simulink library "three_phase_bridge_three_level_ttype_mos_simple_2th"  (R2026a)
settings: Solver=VariableStepAuto
libraries: fl_lib x192, nesl_utility x120, mos_simple_2th_lib x12
(part 2 of 4)

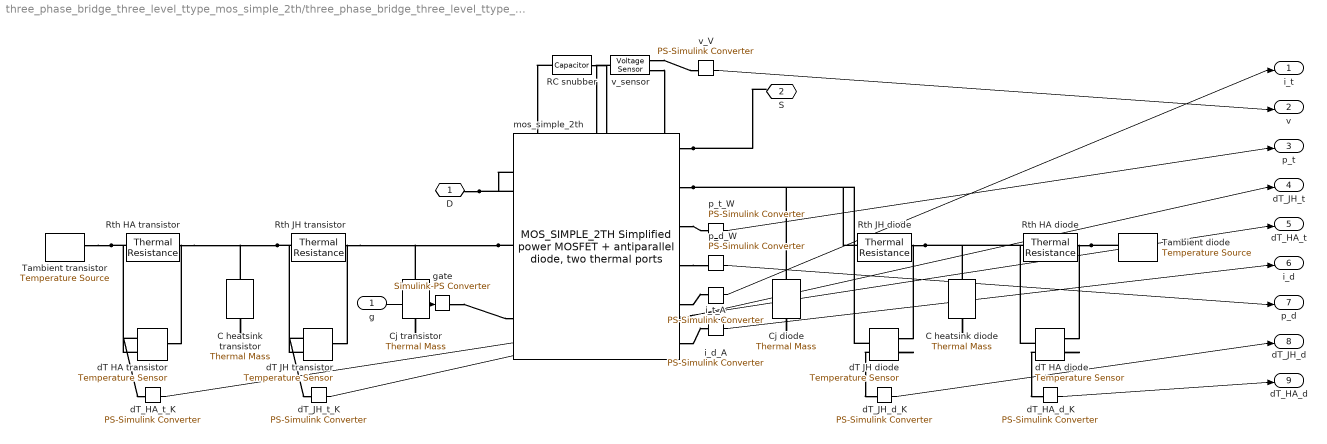
== system three_phase_bridge_three_level_ttype_mos_simple_2th/three_phase_bridge_three_level_ttype_mos_simple_2th/Q4 ==
  g : Inport
  gate : nesl_utility/Simulink-PS Converter  PhysicalDomain=network_engine_domain  SubClassName=ps_input  LeftPortType=input  RightPortType=output  PseudoPeriodic=off  Frequencies=[]  NoiseDistribution=none  NoiseParameters=[]  Unit=1  AffineConversion=off  FilteringAndDerivatives=provide  SimscapeFilterOrder=1  InputFilterTimeConstant=0.001  UdotUserProvided=0
  mos_simple_2th : mos_simple_2th_lib/MOS_SIMPLE_2TH Simplified power MOSFET + antiparallel diode, two thermal ports  Rds_on=rds_on_m mOhm  alpha_R=alpha_R_m 1/K  Tj_ref=Tj_ref_m degC  Roff=Roff_m Ohm  Vf=v_gamma_m V  Rd=rd_on_m mOhm  two_die=two_die_m  G_th=G_th_m  Eon_ref=Eon_m mJ  Eoff_ref=Eoff_m mJ  Err_ref=Err_m mJ  Iref=Ic_ref_m A  Vref=Vdc_ref_m V  ki=ki_m  kv=kv_m  Vth_off=Vth_off_m V  Vth_on=Vth_on_m V  V_sm=V_sm_m V  tau_s=time_constant_edge_m us  tau_v=tau_v_m us  tau_p=time_constant_ploss_m us  i_eps=i_eps_m A  v_eps=1e-3 V  v_specify=off  v_priority=None  v=0 V  v_nominal_specify=off  v_nominal_value=1  v_nominal_unit=V  i_specify=off  i_priority=None  i=0 A  i_nominal_specify=off  i_nominal_value=1  i_nominal_unit=A  ich_specify=off  ich_priority=None  ich=0 A  ich_nominal_specify=off  ich_nominal_value=1  ich_nominal_unit=A  ichp_specify=off  ichp_priority=None  ichp=0 A  ichp_nominal_specify=off  ichp_nominal_value=1  ichp_nominal_unit=A  idio_specify=off  idio_priority=None  idio=0 A  idio_nominal_specify=off  idio_nominal_value=1  idio_nominal_unit=A  vfd_specify=off  vfd_priority=None  vfd=0 V  vfd_nominal_specify=off  vfd_nominal_value=1  vfd_nominal_unit=V  ith_specify=off  ith_priority=None  ith=0 A  ith_nominal_specify=off  ith_nominal_value=1  ith_nominal_unit=A  idh_specify=off  idh_priority=None  idh=0 A  idh_nominal_specify=off  idh_nominal_value=1  idh_nominal_unit=A  vbl_specify=off  vbl_priority=None  vbl=600 V  vbl_nominal_specify=off  vbl_nominal_value=1  vbl_nominal_unit=V  hb_specify=off  hb_priority=None  hb=0  hb_nominal_specify=off  hb_nominal_value=1  hb_nominal_unit=1  Gch_specify=off  Gch_priority=None  Gch=0 S  Gch_nominal_specify=off  Gch_nominal_value=1  Gch_nominal_unit=S  gl_specify=off  gl_priority=None  gl=0  gl_nominal_specify=off  gl_nominal_value=1  gl_nominal_unit=1  Rds_specify=off  Rds_priority=None  Rds=1e-3 Ohm  Rds_nominal_specify=off  Rds_nominal_value=1  Rds_nominal_unit=Ohm  xr_specify=off  xr_priority=None  xr=1  xr_nominal_specify=off  xr_nominal_value=1  xr_nominal_unit=1  Eot_specify=off  Eot_priority=None  Eot=0 J  Eot_nominal_specify=off  Eot_nominal_value=1  Eot_nominal_unit=J  Eod_specify=off  Eod_priority=None  Eod=0 J  Eod_nominal_specify=off  Eod_nominal_value=1  Eod_nominal_unit=J  Pswt_specify=off  Pswt_priority=None  Pswt=0 W  Pswt_nominal_specify=off  Pswt_nominal_value=1  Pswt_nominal_unit=W  Pswd_specify=off  Pswd_priority=None  Pswd=0 W  Pswd_nominal_specify=off  Pswd_nominal_value=1  Pswd_nominal_unit=W  Pct_specify=off  Pct_priority=None  Pct=0 W  Pct_nominal_specify=off  Pct_nominal_value=1  Pct_nominal_unit=W  Pcd_specify=off  Pcd_priority=None  Pcd=0 W  Pcd_nominal_specify=off  Pcd_nominal_value=1  Pcd_nominal_unit=W  Qt_specify=off  Qt_priority=None  Qt=0 W  Qt_nominal_specify=off  Qt_nominal_value=1  Qt_nominal_unit=W  Qd_specify=off  Qd_priority=None  Qd=0 W  Qd_nominal_specify=off  Qd_nominal_value=1  Qd_nominal_unit=W  Eqt_specify=off  Eqt_priority=None  Eqt=0 J  Eqd_specify=off  Eqd_priority=None  Eqd=0 J
  D : PMIOPort  Side=Left
  S : PMIOPort  Port=2  Side=Right
  RC snubber : fl_lib/Electrical/Electrical Elements/Capacitor  c=Csnubber_m F  r=Rsnubber_m Ohm  g=0 1/Ohm  i_specify=off  i_priority=None  i=0 A  i_nominal_specify=off  i_nominal_value=1  i_nominal_unit=A  v_specify=off  v_priority=None  v=0 V  v_nominal_specify=off  v_nominal_value=1  v_nominal_unit=V  vc_specify=off  vc_priority=High  vc=0 V  vc_nominal_specify=off  vc_nominal_value=1  vc_nominal_unit=V
  v_sensor : fl_lib/Electrical/Electrical Sensors/Voltage Sensor
  v_V : nesl_utility/PS-Simulink Converter  PhysicalDomain=network_engine_domain  SubClassName=ps_output  LeftPortType=input  RightPortType=output  PseudoPeriodic=off  Frequencies=[]  VectorFormat=1-D array  Unit=V  AffineConversion=off
  p_t_W : nesl_utility/PS-Simulink Converter  PhysicalDomain=network_engine_domain  SubClassName=ps_output  LeftPortType=input  RightPortType=output  PseudoPeriodic=off  Frequencies=[]  VectorFormat=1-D array  Unit=W  AffineConversion=off
  p_d_W : nesl_utility/PS-Simulink Converter  PhysicalDomain=network_engine_domain  SubClassName=ps_output  LeftPortType=input  RightPortType=output  PseudoPeriodic=off  Frequencies=[]  VectorFormat=1-D array  Unit=W  AffineConversion=off
  i_t_A : nesl_utility/PS-Simulink Converter  PhysicalDomain=network_engine_domain  SubClassName=ps_output  LeftPortType=input  RightPortType=output  PseudoPeriodic=off  Frequencies=[]  VectorFormat=1-D array  Unit=A  AffineConversion=off
  i_d_A : nesl_utility/PS-Simulink Converter  PhysicalDomain=network_engine_domain  SubClassName=ps_output  LeftPortType=input  RightPortType=output  PseudoPeriodic=off  Frequencies=[]  VectorFormat=1-D array  Unit=A  AffineConversion=off
  Cj transistor : fl_lib/Thermal/Thermal Elements/Thermal Mass  mass_type=foundation.enum.constant_variable.constant  mass=JunctionTermalMass_m/specific_heat_m kg  sp_heat=specific_heat_m J/(K*kg)  mass_min=1e-6 kg  num_ports=foundation.enum.numPorts2.one  m_specify=off  m_priority=High  m=1 kg  m_nominal_specify=off  m_nominal_value=1  m_nominal_unit=kg  T_specify=on  T_priority=High  T=Tambient_m degC  T_nominal_specify=off  T_nominal_value=1  T_nominal_unit=K  Q_specify=off  Q_priority=High  Q=0 W  Q_nominal_specify=off  Q_nominal_value=1  Q_nominal_unit=W
  Rth JH transistor : fl_lib/Thermal/Thermal Elements/Thermal Resistance  resistance=rth_switch_JH_m K/W  T_specify=off  T_priority=High  T=0 deltadegC  T_nominal_specify=off  T_nominal_value=1  T_nominal_unit=K  Q_specify=off  Q_priority=None  Q=0 W  Q_nominal_specify=off  Q_nominal_value=1  Q_nominal_unit=W
  C heatsink transistor : fl_lib/Thermal/Thermal Elements/Thermal Mass  mass_type=foundation.enum.constant_variable.constant  mass=mass_heatsink_m kg  sp_heat=specific_heat_m J/(K*kg)  mass_min=1e-6 kg  num_ports=foundation.enum.numPorts2.one  m_specify=off  m_priority=High  m=1 kg  m_nominal_specify=off  m_nominal_value=1  m_nominal_unit=kg  T_specify=on  T_priority=High  T=Tambient_m degC  T_nominal_specify=off  T_nominal_value=1  T_nominal_unit=K  Q_specify=off  Q_priority=High  Q=0 W  Q_nominal_specify=off  Q_nominal_value=1  Q_nominal_unit=W
  Rth HA transistor : fl_lib/Thermal/Thermal Elements/Thermal Resistance  resistance=rth_switch_HA_m K/W  T_specify=off  T_priority=High  T=0 deltadegC  T_nominal_specify=off  T_nominal_value=1  T_nominal_unit=K  Q_specify=off  Q_priority=None  Q=0 W  Q_nominal_specify=off  Q_nominal_value=1  Q_nominal_unit=W
  Tambient transistor : fl_lib/Thermal/Thermal Sources/Temperature Source  temperature=Tambient_m degC
  dT JH transistor : fl_lib/Thermal/Thermal Sensors/Temperature Sensor  temperature_measure=foundation.enum.MeasurementReference.difference
  dT HA transistor : fl_lib/Thermal/Thermal Sensors/Temperature Sensor  temperature_measure=foundation.enum.MeasurementReference.difference
  dT_JH_t_K : nesl_utility/PS-Simulink Converter  PhysicalDomain=network_engine_domain  SubClassName=ps_output  LeftPortType=input  RightPortType=output  PseudoPeriodic=off  Frequencies=[]  VectorFormat=1-D array  Unit=K  AffineConversion=off
  dT_HA_t_K : nesl_utility/PS-Simulink Converter  PhysicalDomain=network_engine_domain  SubClassName=ps_output  LeftPortType=input  RightPortType=output  PseudoPeriodic=off  Frequencies=[]  VectorFormat=1-D array  Unit=K  AffineConversion=off
  Cj diode : fl_lib/Thermal/Thermal Elements/Thermal Mass  mass_type=foundation.enum.constant_variable.constant  mass=JunctionTermalMass_m/specific_heat_m kg  sp_heat=specific_heat_m J/(K*kg)  mass_min=1e-6 kg  num_ports=foundation.enum.numPorts2.one  m_specify=off  m_priority=High  m=1 kg  m_nominal_specify=off  m_nominal_value=1  m_nominal_unit=kg  T_specify=on  T_priority=High  T=Tambient_m degC  T_nominal_specify=off  T_nominal_value=1  T_nominal_unit=K  Q_specify=off  Q_priority=High  Q=0 W  Q_nominal_specify=off  Q_nominal_value=1  Q_nominal_unit=W
  Rth JH diode : fl_lib/Thermal/Thermal Elements/Thermal Resistance  resistance=rth_diode_JH_m K/W  T_specify=off  T_priority=High  T=0 deltadegC  T_nominal_specify=off  T_nominal_value=1  T_nominal_unit=K  Q_specify=off  Q_priority=None  Q=0 W  Q_nominal_specify=off  Q_nominal_value=1  Q_nominal_unit=W
  C heatsink diode : fl_lib/Thermal/Thermal Elements/Thermal Mass  mass_type=foundation.enum.constant_variable.constant  mass=mass_heatsink_m kg  sp_heat=specific_heat_m J/(K*kg)  mass_min=1e-6 kg  num_ports=foundation.enum.numPorts2.one  m_specify=off  m_priority=High  m=1 kg  m_nominal_specify=off  m_nominal_value=1  m_nominal_unit=kg  T_specify=on  T_priority=High  T=Tambient_m degC  T_nominal_specify=off  T_nominal_value=1  T_nominal_unit=K  Q_specify=off  Q_priority=High  Q=0 W  Q_nominal_specify=off  Q_nominal_value=1  Q_nominal_unit=W
  Rth HA diode : fl_lib/Thermal/Thermal Elements/Thermal Resistance  resistance=rth_diode_HA_m K/W  T_specify=off  T_priority=High  T=0 deltadegC  T_nominal_specify=off  T_nominal_value=1  T_nominal_unit=K  Q_specify=off  Q_priority=None  Q=0 W  Q_nominal_specify=off  Q_nominal_value=1  Q_nominal_unit=W
  Tambient diode : fl_lib/Thermal/Thermal Sources/Temperature Source  temperature=Tambient_m degC
  dT JH diode : fl_lib/Thermal/Thermal Sensors/Temperature Sensor  temperature_measure=foundation.enum.MeasurementReference.difference
  dT HA diode : fl_lib/Thermal/Thermal Sensors/Temperature Sensor  temperature_measure=foundation.enum.MeasurementReference.difference
  dT_JH_d_K : nesl_utility/PS-Simulink Converter  PhysicalDomain=network_engine_domain  SubClassName=ps_output  LeftPortType=input  RightPortType=output  PseudoPeriodic=off  Frequencies=[]  VectorFormat=1-D array  Unit=K  AffineConversion=off
  dT_HA_d_K : nesl_utility/PS-Simulink Converter  PhysicalDomain=network_engine_domain  SubClassName=ps_output  LeftPortType=input  RightPortType=output  PseudoPeriodic=off  Frequencies=[]  VectorFormat=1-D array  Unit=K  AffineConversion=off
  i_t : Outport
  v : Outport  Port=2
  p_t : Outport  Port=3
  dT_JH_t : Outport  Port=4
  dT_HA_t : Outport  Port=5
  i_d : Outport  Port=6
  p_d : Outport  Port=7
  dT_JH_d : Outport  Port=8
  dT_HA_d : Outport  Port=9
  wires:
  i_t_A/1 -> i_t/1
  v_V/1 -> v/1
  p_t_W/1 -> p_t/1
  dT_JH_t_K/1 -> dT_JH_t/1
  dT_HA_t_K/1 -> dT_HA_t/1
  i_d_A/1 -> i_d/1
  p_d_W/1 -> p_d/1
  dT_JH_d_K/1 -> dT_JH_d/1
  dT_HA_d_K/1 -> dT_HA_d/1
  g/1 -> gate/1
  connections:
  Rth JH transistor/RConn1 -- C heatsink transistor/LConn1 -- Rth HA transistor/LConn1 -- dT JH transistor/RConn1 -- dT HA transistor/LConn1
  Rth HA transistor/RConn1 -- Tambient transistor/LConn1 -- dT HA transistor/RConn1
  dT JH transistor/RConn2 -- dT_JH_t_K/LConn1
  dT HA transistor/RConn2 -- dT_HA_t_K/LConn1
  Rth JH diode/RConn1 -- C heatsink diode/LConn1 -- Rth HA diode/LConn1 -- dT JH diode/RConn1 -- dT HA diode/LConn1
  Rth HA diode/RConn1 -- Tambient diode/LConn1 -- dT HA diode/RConn1
  dT JH diode/RConn2 -- dT_JH_d_K/LConn1
  dT HA diode/RConn2 -- dT_HA_d_K/LConn1
  gate/RConn1 -- mos_simple_2th/LConn3
  D/RConn1 -- mos_simple_2th/LConn1 -- RC snubber/LConn1 -- v_sensor/LConn1
  mos_simple_2th/RConn1 -- S/RConn1 -- RC snubber/RConn1 -- v_sensor/RConn2
  v_sensor/RConn1 -- v_V/LConn1
  mos_simple_2th/RConn3 -- p_t_W/LConn1
  mos_simple_2th/RConn4 -- p_d_W/LConn1
  mos_simple_2th/RConn5 -- i_t_A/LConn1
  mos_simple_2th/RConn6 -- i_d_A/LConn1
  mos_simple_2th/LConn2 -- Cj transistor/LConn1 -- Rth JH transistor/LConn1 -- dT JH transistor/LConn1
  mos_simple_2th/RConn2 -- Cj diode/LConn1 -- Rth JH diode/LConn1 -- dT JH diode/LConn1

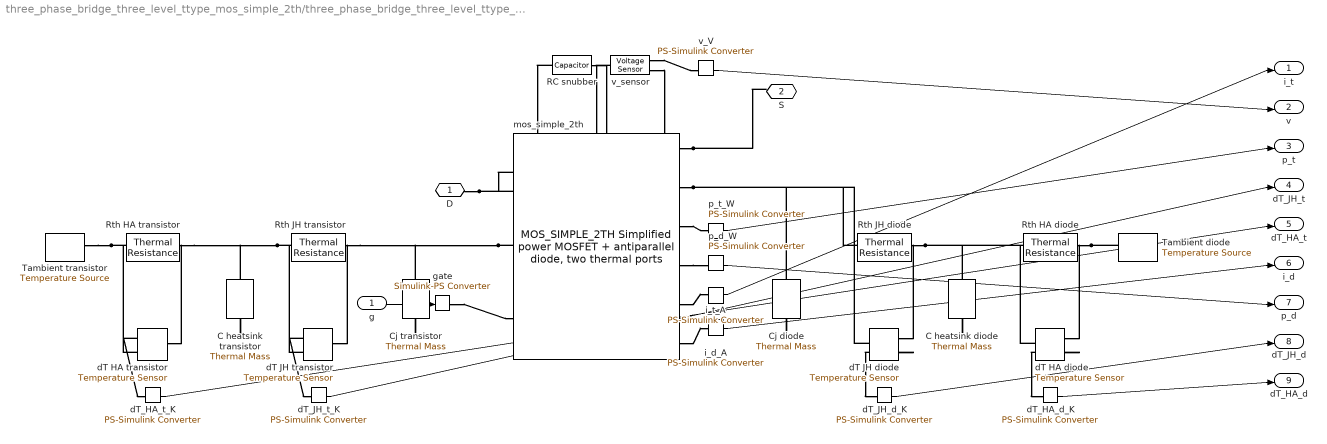
== system three_phase_bridge_three_level_ttype_mos_simple_2th/three_phase_bridge_three_level_ttype_mos_simple_2th/Q5 ==
  g : Inport
  gate : nesl_utility/Simulink-PS Converter  PhysicalDomain=network_engine_domain  SubClassName=ps_input  LeftPortType=input  RightPortType=output  PseudoPeriodic=off  Frequencies=[]  NoiseDistribution=none  NoiseParameters=[]  Unit=1  AffineConversion=off  FilteringAndDerivatives=provide  SimscapeFilterOrder=1  InputFilterTimeConstant=0.001  UdotUserProvided=0
  mos_simple_2th : mos_simple_2th_lib/MOS_SIMPLE_2TH Simplified power MOSFET + antiparallel diode, two thermal ports  Rds_on=rds_on_m mOhm  alpha_R=alpha_R_m 1/K  Tj_ref=Tj_ref_m degC  Roff=Roff_m Ohm  Vf=v_gamma_m V  Rd=rd_on_m mOhm  two_die=two_die_m  G_th=G_th_m  Eon_ref=Eon_m mJ  Eoff_ref=Eoff_m mJ  Err_ref=Err_m mJ  Iref=Ic_ref_m A  Vref=Vdc_ref_m V  ki=ki_m  kv=kv_m  Vth_off=Vth_off_m V  Vth_on=Vth_on_m V  V_sm=V_sm_m V  tau_s=time_constant_edge_m us  tau_v=tau_v_m us  tau_p=time_constant_ploss_m us  i_eps=i_eps_m A  v_eps=1e-3 V  v_specify=off  v_priority=None  v=0 V  v_nominal_specify=off  v_nominal_value=1  v_nominal_unit=V  i_specify=off  i_priority=None  i=0 A  i_nominal_specify=off  i_nominal_value=1  i_nominal_unit=A  ich_specify=off  ich_priority=None  ich=0 A  ich_nominal_specify=off  ich_nominal_value=1  ich_nominal_unit=A  ichp_specify=off  ichp_priority=None  ichp=0 A  ichp_nominal_specify=off  ichp_nominal_value=1  ichp_nominal_unit=A  idio_specify=off  idio_priority=None  idio=0 A  idio_nominal_specify=off  idio_nominal_value=1  idio_nominal_unit=A  vfd_specify=off  vfd_priority=None  vfd=0 V  vfd_nominal_specify=off  vfd_nominal_value=1  vfd_nominal_unit=V  ith_specify=off  ith_priority=None  ith=0 A  ith_nominal_specify=off  ith_nominal_value=1  ith_nominal_unit=A  idh_specify=off  idh_priority=None  idh=0 A  idh_nominal_specify=off  idh_nominal_value=1  idh_nominal_unit=A  vbl_specify=off  vbl_priority=None  vbl=600 V  vbl_nominal_specify=off  vbl_nominal_value=1  vbl_nominal_unit=V  hb_specify=off  hb_priority=None  hb=0  hb_nominal_specify=off  hb_nominal_value=1  hb_nominal_unit=1  Gch_specify=off  Gch_priority=None  Gch=0 S  Gch_nominal_specify=off  Gch_nominal_value=1  Gch_nominal_unit=S  gl_specify=off  gl_priority=None  gl=0  gl_nominal_specify=off  gl_nominal_value=1  gl_nominal_unit=1  Rds_specify=off  Rds_priority=None  Rds=1e-3 Ohm  Rds_nominal_specify=off  Rds_nominal_value=1  Rds_nominal_unit=Ohm  xr_specify=off  xr_priority=None  xr=1  xr_nominal_specify=off  xr_nominal_value=1  xr_nominal_unit=1  Eot_specify=off  Eot_priority=None  Eot=0 J  Eot_nominal_specify=off  Eot_nominal_value=1  Eot_nominal_unit=J  Eod_specify=off  Eod_priority=None  Eod=0 J  Eod_nominal_specify=off  Eod_nominal_value=1  Eod_nominal_unit=J  Pswt_specify=off  Pswt_priority=None  Pswt=0 W  Pswt_nominal_specify=off  Pswt_nominal_value=1  Pswt_nominal_unit=W  Pswd_specify=off  Pswd_priority=None  Pswd=0 W  Pswd_nominal_specify=off  Pswd_nominal_value=1  Pswd_nominal_unit=W  Pct_specify=off  Pct_priority=None  Pct=0 W  Pct_nominal_specify=off  Pct_nominal_value=1  Pct_nominal_unit=W  Pcd_specify=off  Pcd_priority=None  Pcd=0 W  Pcd_nominal_specify=off  Pcd_nominal_value=1  Pcd_nominal_unit=W  Qt_specify=off  Qt_priority=None  Qt=0 W  Qt_nominal_specify=off  Qt_nominal_value=1  Qt_nominal_unit=W  Qd_specify=off  Qd_priority=None  Qd=0 W  Qd_nominal_specify=off  Qd_nominal_value=1  Qd_nominal_unit=W  Eqt_specify=off  Eqt_priority=None  Eqt=0 J  Eqd_specify=off  Eqd_priority=None  Eqd=0 J
  D : PMIOPort  Side=Left
  S : PMIOPort  Port=2  Side=Right
  RC snubber : fl_lib/Electrical/Electrical Elements/Capacitor  c=Csnubber_m F  r=Rsnubber_m Ohm  g=0 1/Ohm  i_specify=off  i_priority=None  i=0 A  i_nominal_specify=off  i_nominal_value=1  i_nominal_unit=A  v_specify=off  v_priority=None  v=0 V  v_nominal_specify=off  v_nominal_value=1  v_nominal_unit=V  vc_specify=off  vc_priority=High  vc=0 V  vc_nominal_specify=off  vc_nominal_value=1  vc_nominal_unit=V
  v_sensor : fl_lib/Electrical/Electrical Sensors/Voltage Sensor
  v_V : nesl_utility/PS-Simulink Converter  PhysicalDomain=network_engine_domain  SubClassName=ps_output  LeftPortType=input  RightPortType=output  PseudoPeriodic=off  Frequencies=[]  VectorFormat=1-D array  Unit=V  AffineConversion=off
  p_t_W : nesl_utility/PS-Simulink Converter  PhysicalDomain=network_engine_domain  SubClassName=ps_output  LeftPortType=input  RightPortType=output  PseudoPeriodic=off  Frequencies=[]  VectorFormat=1-D array  Unit=W  AffineConversion=off
  p_d_W : nesl_utility/PS-Simulink Converter  PhysicalDomain=network_engine_domain  SubClassName=ps_output  LeftPortType=input  RightPortType=output  PseudoPeriodic=off  Frequencies=[]  VectorFormat=1-D array  Unit=W  AffineConversion=off
  i_t_A : nesl_utility/PS-Simulink Converter  PhysicalDomain=network_engine_domain  SubClassName=ps_output  LeftPortType=input  RightPortType=output  PseudoPeriodic=off  Frequencies=[]  VectorFormat=1-D array  Unit=A  AffineConversion=off
  i_d_A : nesl_utility/PS-Simulink Converter  PhysicalDomain=network_engine_domain  SubClassName=ps_output  LeftPortType=input  RightPortType=output  PseudoPeriodic=off  Frequencies=[]  VectorFormat=1-D array  Unit=A  AffineConversion=off
  Cj transistor : fl_lib/Thermal/Thermal Elements/Thermal Mass  mass_type=foundation.enum.constant_variable.constant  mass=JunctionTermalMass_m/specific_heat_m kg  sp_heat=specific_heat_m J/(K*kg)  mass_min=1e-6 kg  num_ports=foundation.enum.numPorts2.one  m_specify=off  m_priority=High  m=1 kg  m_nominal_specify=off  m_nominal_value=1  m_nominal_unit=kg  T_specify=on  T_priority=High  T=Tambient_m degC  T_nominal_specify=off  T_nominal_value=1  T_nominal_unit=K  Q_specify=off  Q_priority=High  Q=0 W  Q_nominal_specify=off  Q_nominal_value=1  Q_nominal_unit=W
  Rth JH transistor : fl_lib/Thermal/Thermal Elements/Thermal Resistance  resistance=rth_switch_JH_m K/W  T_specify=off  T_priority=High  T=0 deltadegC  T_nominal_specify=off  T_nominal_value=1  T_nominal_unit=K  Q_specify=off  Q_priority=None  Q=0 W  Q_nominal_specify=off  Q_nominal_value=1  Q_nominal_unit=W
  C heatsink transistor : fl_lib/Thermal/Thermal Elements/Thermal Mass  mass_type=foundation.enum.constant_variable.constant  mass=mass_heatsink_m kg  sp_heat=specific_heat_m J/(K*kg)  mass_min=1e-6 kg  num_ports=foundation.enum.numPorts2.one  m_specify=off  m_priority=High  m=1 kg  m_nominal_specify=off  m_nominal_value=1  m_nominal_unit=kg  T_specify=on  T_priority=High  T=Tambient_m degC  T_nominal_specify=off  T_nominal_value=1  T_nominal_unit=K  Q_specify=off  Q_priority=High  Q=0 W  Q_nominal_specify=off  Q_nominal_value=1  Q_nominal_unit=W
  Rth HA transistor : fl_lib/Thermal/Thermal Elements/Thermal Resistance  resistance=rth_switch_HA_m K/W  T_specify=off  T_priority=High  T=0 deltadegC  T_nominal_specify=off  T_nominal_value=1  T_nominal_unit=K  Q_specify=off  Q_priority=None  Q=0 W  Q_nominal_specify=off  Q_nominal_value=1  Q_nominal_unit=W
  Tambient transistor : fl_lib/Thermal/Thermal Sources/Temperature Source  temperature=Tambient_m degC
  dT JH transistor : fl_lib/Thermal/Thermal Sensors/Temperature Sensor  temperature_measure=foundation.enum.MeasurementReference.difference
  dT HA transistor : fl_lib/Thermal/Thermal Sensors/Temperature Sensor  temperature_measure=foundation.enum.MeasurementReference.difference
  dT_JH_t_K : nesl_utility/PS-Simulink Converter  PhysicalDomain=network_engine_domain  SubClassName=ps_output  LeftPortType=input  RightPortType=output  PseudoPeriodic=off  Frequencies=[]  VectorFormat=1-D array  Unit=K  AffineConversion=off
  dT_HA_t_K : nesl_utility/PS-Simulink Converter  PhysicalDomain=network_engine_domain  SubClassName=ps_output  LeftPortType=input  RightPortType=output  PseudoPeriodic=off  Frequencies=[]  VectorFormat=1-D array  Unit=K  AffineConversion=off
  Cj diode : fl_lib/Thermal/Thermal Elements/Thermal Mass  mass_type=foundation.enum.constant_variable.constant  mass=JunctionTermalMass_m/specific_heat_m kg  sp_heat=specific_heat_m J/(K*kg)  mass_min=1e-6 kg  num_ports=foundation.enum.numPorts2.one  m_specify=off  m_priority=High  m=1 kg  m_nominal_specify=off  m_nominal_value=1  m_nominal_unit=kg  T_specify=on  T_priority=High  T=Tambient_m degC  T_nominal_specify=off  T_nominal_value=1  T_nominal_unit=K  Q_specify=off  Q_priority=High  Q=0 W  Q_nominal_specify=off  Q_nominal_value=1  Q_nominal_unit=W
  Rth JH diode : fl_lib/Thermal/Thermal Elements/Thermal Resistance  resistance=rth_diode_JH_m K/W  T_specify=off  T_priority=High  T=0 deltadegC  T_nominal_specify=off  T_nominal_value=1  T_nominal_unit=K  Q_specify=off  Q_priority=None  Q=0 W  Q_nominal_specify=off  Q_nominal_value=1  Q_nominal_unit=W
  C heatsink diode : fl_lib/Thermal/Thermal Elements/Thermal Mass  mass_type=foundation.enum.constant_variable.constant  mass=mass_heatsink_m kg  sp_heat=specific_heat_m J/(K*kg)  mass_min=1e-6 kg  num_ports=foundation.enum.numPorts2.one  m_specify=off  m_priority=High  m=1 kg  m_nominal_specify=off  m_nominal_value=1  m_nominal_unit=kg  T_specify=on  T_priority=High  T=Tambient_m degC  T_nominal_specify=off  T_nominal_value=1  T_nominal_unit=K  Q_specify=off  Q_priority=High  Q=0 W  Q_nominal_specify=off  Q_nominal_value=1  Q_nominal_unit=W
  Rth HA diode : fl_lib/Thermal/Thermal Elements/Thermal Resistance  resistance=rth_diode_HA_m K/W  T_specify=off  T_priority=High  T=0 deltadegC  T_nominal_specify=off  T_nominal_value=1  T_nominal_unit=K  Q_specify=off  Q_priority=None  Q=0 W  Q_nominal_specify=off  Q_nominal_value=1  Q_nominal_unit=W
  Tambient diode : fl_lib/Thermal/Thermal Sources/Temperature Source  temperature=Tambient_m degC
  dT JH diode : fl_lib/Thermal/Thermal Sensors/Temperature Sensor  temperature_measure=foundation.enum.MeasurementReference.difference
  dT HA diode : fl_lib/Thermal/Thermal Sensors/Temperature Sensor  temperature_measure=foundation.enum.MeasurementReference.difference
  dT_JH_d_K : nesl_utility/PS-Simulink Converter  PhysicalDomain=network_engine_domain  SubClassName=ps_output  LeftPortType=input  RightPortType=output  PseudoPeriodic=off  Frequencies=[]  VectorFormat=1-D array  Unit=K  AffineConversion=off
  dT_HA_d_K : nesl_utility/PS-Simulink Converter  PhysicalDomain=network_engine_domain  SubClassName=ps_output  LeftPortType=input  RightPortType=output  PseudoPeriodic=off  Frequencies=[]  VectorFormat=1-D array  Unit=K  AffineConversion=off
  i_t : Outport
  v : Outport  Port=2
  p_t : Outport  Port=3
  dT_JH_t : Outport  Port=4
  dT_HA_t : Outport  Port=5
  i_d : Outport  Port=6
  p_d : Outport  Port=7
  dT_JH_d : Outport  Port=8
  dT_HA_d : Outport  Port=9
  wires:
  i_t_A/1 -> i_t/1
  v_V/1 -> v/1
  p_t_W/1 -> p_t/1
  dT_JH_t_K/1 -> dT_JH_t/1
  dT_HA_t_K/1 -> dT_HA_t/1
  i_d_A/1 -> i_d/1
  p_d_W/1 -> p_d/1
  dT_JH_d_K/1 -> dT_JH_d/1
  dT_HA_d_K/1 -> dT_HA_d/1
  g/1 -> gate/1
  connections:
  Rth JH transistor/RConn1 -- C heatsink transistor/LConn1 -- Rth HA transistor/LConn1 -- dT JH transistor/RConn1 -- dT HA transistor/LConn1
  Rth HA transistor/RConn1 -- Tambient transistor/LConn1 -- dT HA transistor/RConn1
  dT JH transistor/RConn2 -- dT_JH_t_K/LConn1
  dT HA transistor/RConn2 -- dT_HA_t_K/LConn1
  Rth JH diode/RConn1 -- C heatsink diode/LConn1 -- Rth HA diode/LConn1 -- dT JH diode/RConn1 -- dT HA diode/LConn1
  Rth HA diode/RConn1 -- Tambient diode/LConn1 -- dT HA diode/RConn1
  dT JH diode/RConn2 -- dT_JH_d_K/LConn1
  dT HA diode/RConn2 -- dT_HA_d_K/LConn1
  gate/RConn1 -- mos_simple_2th/LConn3
  D/RConn1 -- mos_simple_2th/LConn1 -- RC snubber/LConn1 -- v_sensor/LConn1
  mos_simple_2th/RConn1 -- S/RConn1 -- RC snubber/RConn1 -- v_sensor/RConn2
  v_sensor/RConn1 -- v_V/LConn1
  mos_simple_2th/RConn3 -- p_t_W/LConn1
  mos_simple_2th/RConn4 -- p_d_W/LConn1
  mos_simple_2th/RConn5 -- i_t_A/LConn1
  mos_simple_2th/RConn6 -- i_d_A/LConn1
  mos_simple_2th/LConn2 -- Cj transistor/LConn1 -- Rth JH transistor/LConn1 -- dT JH transistor/LConn1
  mos_simple_2th/RConn2 -- Cj diode/LConn1 -- Rth JH diode/LConn1 -- dT JH diode/LConn1

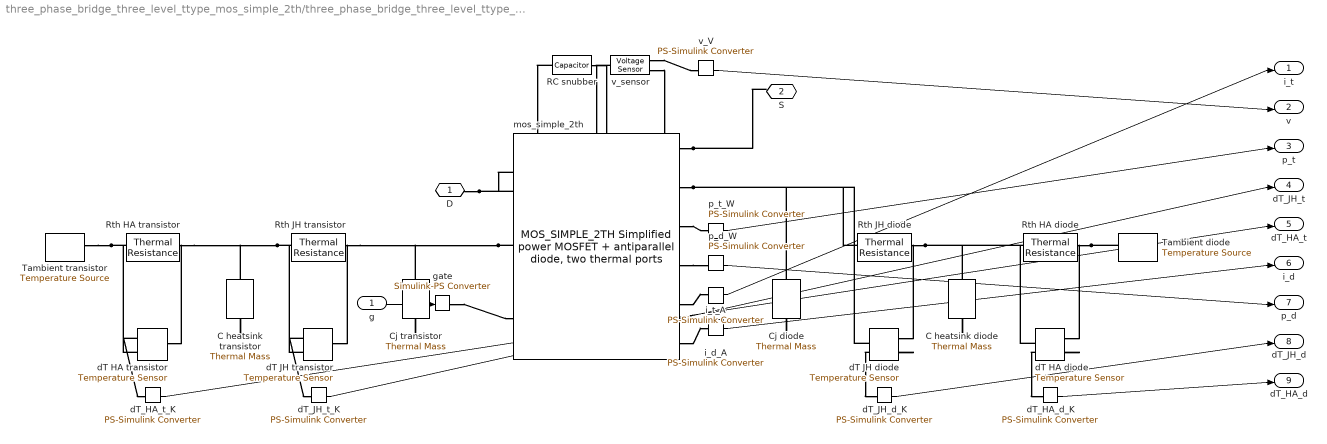
== system three_phase_bridge_three_level_ttype_mos_simple_2th/three_phase_bridge_three_level_ttype_mos_simple_2th/Q6 ==
  g : Inport
  gate : nesl_utility/Simulink-PS Converter  PhysicalDomain=network_engine_domain  SubClassName=ps_input  LeftPortType=input  RightPortType=output  PseudoPeriodic=off  Frequencies=[]  NoiseDistribution=none  NoiseParameters=[]  Unit=1  AffineConversion=off  FilteringAndDerivatives=provide  SimscapeFilterOrder=1  InputFilterTimeConstant=0.001  UdotUserProvided=0
  mos_simple_2th : mos_simple_2th_lib/MOS_SIMPLE_2TH Simplified power MOSFET + antiparallel diode, two thermal ports  Rds_on=rds_on_m mOhm  alpha_R=alpha_R_m 1/K  Tj_ref=Tj_ref_m degC  Roff=Roff_m Ohm  Vf=v_gamma_m V  Rd=rd_on_m mOhm  two_die=two_die_m  G_th=G_th_m  Eon_ref=Eon_m mJ  Eoff_ref=Eoff_m mJ  Err_ref=Err_m mJ  Iref=Ic_ref_m A  Vref=Vdc_ref_m V  ki=ki_m  kv=kv_m  Vth_off=Vth_off_m V  Vth_on=Vth_on_m V  V_sm=V_sm_m V  tau_s=time_constant_edge_m us  tau_v=tau_v_m us  tau_p=time_constant_ploss_m us  i_eps=i_eps_m A  v_eps=1e-3 V  v_specify=off  v_priority=None  v=0 V  v_nominal_specify=off  v_nominal_value=1  v_nominal_unit=V  i_specify=off  i_priority=None  i=0 A  i_nominal_specify=off  i_nominal_value=1  i_nominal_unit=A  ich_specify=off  ich_priority=None  ich=0 A  ich_nominal_specify=off  ich_nominal_value=1  ich_nominal_unit=A  ichp_specify=off  ichp_priority=None  ichp=0 A  ichp_nominal_specify=off  ichp_nominal_value=1  ichp_nominal_unit=A  idio_specify=off  idio_priority=None  idio=0 A  idio_nominal_specify=off  idio_nominal_value=1  idio_nominal_unit=A  vfd_specify=off  vfd_priority=None  vfd=0 V  vfd_nominal_specify=off  vfd_nominal_value=1  vfd_nominal_unit=V  ith_specify=off  ith_priority=None  ith=0 A  ith_nominal_specify=off  ith_nominal_value=1  ith_nominal_unit=A  idh_specify=off  idh_priority=None  idh=0 A  idh_nominal_specify=off  idh_nominal_value=1  idh_nominal_unit=A  vbl_specify=off  vbl_priority=None  vbl=600 V  vbl_nominal_specify=off  vbl_nominal_value=1  vbl_nominal_unit=V  hb_specify=off  hb_priority=None  hb=0  hb_nominal_specify=off  hb_nominal_value=1  hb_nominal_unit=1  Gch_specify=off  Gch_priority=None  Gch=0 S  Gch_nominal_specify=off  Gch_nominal_value=1  Gch_nominal_unit=S  gl_specify=off  gl_priority=None  gl=0  gl_nominal_specify=off  gl_nominal_value=1  gl_nominal_unit=1  Rds_specify=off  Rds_priority=None  Rds=1e-3 Ohm  Rds_nominal_specify=off  Rds_nominal_value=1  Rds_nominal_unit=Ohm  xr_specify=off  xr_priority=None  xr=1  xr_nominal_specify=off  xr_nominal_value=1  xr_nominal_unit=1  Eot_specify=off  Eot_priority=None  Eot=0 J  Eot_nominal_specify=off  Eot_nominal_value=1  Eot_nominal_unit=J  Eod_specify=off  Eod_priority=None  Eod=0 J  Eod_nominal_specify=off  Eod_nominal_value=1  Eod_nominal_unit=J  Pswt_specify=off  Pswt_priority=None  Pswt=0 W  Pswt_nominal_specify=off  Pswt_nominal_value=1  Pswt_nominal_unit=W  Pswd_specify=off  Pswd_priority=None  Pswd=0 W  Pswd_nominal_specify=off  Pswd_nominal_value=1  Pswd_nominal_unit=W  Pct_specify=off  Pct_priority=None  Pct=0 W  Pct_nominal_specify=off  Pct_nominal_value=1  Pct_nominal_unit=W  Pcd_specify=off  Pcd_priority=None  Pcd=0 W  Pcd_nominal_specify=off  Pcd_nominal_value=1  Pcd_nominal_unit=W  Qt_specify=off  Qt_priority=None  Qt=0 W  Qt_nominal_specify=off  Qt_nominal_value=1  Qt_nominal_unit=W  Qd_specify=off  Qd_priority=None  Qd=0 W  Qd_nominal_specify=off  Qd_nominal_value=1  Qd_nominal_unit=W  Eqt_specify=off  Eqt_priority=None  Eqt=0 J  Eqd_specify=off  Eqd_priority=None  Eqd=0 J
  D : PMIOPort  Side=Left
  S : PMIOPort  Port=2  Side=Right
  RC snubber : fl_lib/Electrical/Electrical Elements/Capacitor  c=Csnubber_m F  r=Rsnubber_m Ohm  g=0 1/Ohm  i_specify=off  i_priority=None  i=0 A  i_nominal_specify=off  i_nominal_value=1  i_nominal_unit=A  v_specify=off  v_priority=None  v=0 V  v_nominal_specify=off  v_nominal_value=1  v_nominal_unit=V  vc_specify=off  vc_priority=High  vc=0 V  vc_nominal_specify=off  vc_nominal_value=1  vc_nominal_unit=V
  v_sensor : fl_lib/Electrical/Electrical Sensors/Voltage Sensor
  v_V : nesl_utility/PS-Simulink Converter  PhysicalDomain=network_engine_domain  SubClassName=ps_output  LeftPortType=input  RightPortType=output  PseudoPeriodic=off  Frequencies=[]  VectorFormat=1-D array  Unit=V  AffineConversion=off
  p_t_W : nesl_utility/PS-Simulink Converter  PhysicalDomain=network_engine_domain  SubClassName=ps_output  LeftPortType=input  RightPortType=output  PseudoPeriodic=off  Frequencies=[]  VectorFormat=1-D array  Unit=W  AffineConversion=off
  p_d_W : nesl_utility/PS-Simulink Converter  PhysicalDomain=network_engine_domain  SubClassName=ps_output  LeftPortType=input  RightPortType=output  PseudoPeriodic=off  Frequencies=[]  VectorFormat=1-D array  Unit=W  AffineConversion=off
  i_t_A : nesl_utility/PS-Simulink Converter  PhysicalDomain=network_engine_domain  SubClassName=ps_output  LeftPortType=input  RightPortType=output  PseudoPeriodic=off  Frequencies=[]  VectorFormat=1-D array  Unit=A  AffineConversion=off
  i_d_A : nesl_utility/PS-Simulink Converter  PhysicalDomain=network_engine_domain  SubClassName=ps_output  LeftPortType=input  RightPortType=output  PseudoPeriodic=off  Frequencies=[]  VectorFormat=1-D array  Unit=A  AffineConversion=off
  Cj transistor : fl_lib/Thermal/Thermal Elements/Thermal Mass  mass_type=foundation.enum.constant_variable.constant  mass=JunctionTermalMass_m/specific_heat_m kg  sp_heat=specific_heat_m J/(K*kg)  mass_min=1e-6 kg  num_ports=foundation.enum.numPorts2.one  m_specify=off  m_priority=High  m=1 kg  m_nominal_specify=off  m_nominal_value=1  m_nominal_unit=kg  T_specify=on  T_priority=High  T=Tambient_m degC  T_nominal_specify=off  T_nominal_value=1  T_nominal_unit=K  Q_specify=off  Q_priority=High  Q=0 W  Q_nominal_specify=off  Q_nominal_value=1  Q_nominal_unit=W
  Rth JH transistor : fl_lib/Thermal/Thermal Elements/Thermal Resistance  resistance=rth_switch_JH_m K/W  T_specify=off  T_priority=High  T=0 deltadegC  T_nominal_specify=off  T_nominal_value=1  T_nominal_unit=K  Q_specify=off  Q_priority=None  Q=0 W  Q_nominal_specify=off  Q_nominal_value=1  Q_nominal_unit=W
  C heatsink transistor : fl_lib/Thermal/Thermal Elements/Thermal Mass  mass_type=foundation.enum.constant_variable.constant  mass=mass_heatsink_m kg  sp_heat=specific_heat_m J/(K*kg)  mass_min=1e-6 kg  num_ports=foundation.enum.numPorts2.one  m_specify=off  m_priority=High  m=1 kg  m_nominal_specify=off  m_nominal_value=1  m_nominal_unit=kg  T_specify=on  T_priority=High  T=Tambient_m degC  T_nominal_specify=off  T_nominal_value=1  T_nominal_unit=K  Q_specify=off  Q_priority=High  Q=0 W  Q_nominal_specify=off  Q_nominal_value=1  Q_nominal_unit=W
  Rth HA transistor : fl_lib/Thermal/Thermal Elements/Thermal Resistance  resistance=rth_switch_HA_m K/W  T_specify=off  T_priority=High  T=0 deltadegC  T_nominal_specify=off  T_nominal_value=1  T_nominal_unit=K  Q_specify=off  Q_priority=None  Q=0 W  Q_nominal_specify=off  Q_nominal_value=1  Q_nominal_unit=W
  Tambient transistor : fl_lib/Thermal/Thermal Sources/Temperature Source  temperature=Tambient_m degC
  dT JH transistor : fl_lib/Thermal/Thermal Sensors/Temperature Sensor  temperature_measure=foundation.enum.MeasurementReference.difference
  dT HA transistor : fl_lib/Thermal/Thermal Sensors/Temperature Sensor  temperature_measure=foundation.enum.MeasurementReference.difference
  dT_JH_t_K : nesl_utility/PS-Simulink Converter  PhysicalDomain=network_engine_domain  SubClassName=ps_output  LeftPortType=input  RightPortType=output  PseudoPeriodic=off  Frequencies=[]  VectorFormat=1-D array  Unit=K  AffineConversion=off
  dT_HA_t_K : nesl_utility/PS-Simulink Converter  PhysicalDomain=network_engine_domain  SubClassName=ps_output  LeftPortType=input  RightPortType=output  PseudoPeriodic=off  Frequencies=[]  VectorFormat=1-D array  Unit=K  AffineConversion=off
  Cj diode : fl_lib/Thermal/Thermal Elements/Thermal Mass  mass_type=foundation.enum.constant_variable.constant  mass=JunctionTermalMass_m/specific_heat_m kg  sp_heat=specific_heat_m J/(K*kg)  mass_min=1e-6 kg  num_ports=foundation.enum.numPorts2.one  m_specify=off  m_priority=High  m=1 kg  m_nominal_specify=off  m_nominal_value=1  m_nominal_unit=kg  T_specify=on  T_priority=High  T=Tambient_m degC  T_nominal_specify=off  T_nominal_value=1  T_nominal_unit=K  Q_specify=off  Q_priority=High  Q=0 W  Q_nominal_specify=off  Q_nominal_value=1  Q_nominal_unit=W
  Rth JH diode : fl_lib/Thermal/Thermal Elements/Thermal Resistance  resistance=rth_diode_JH_m K/W  T_specify=off  T_priority=High  T=0 deltadegC  T_nominal_specify=off  T_nominal_value=1  T_nominal_unit=K  Q_specify=off  Q_priority=None  Q=0 W  Q_nominal_specify=off  Q_nominal_value=1  Q_nominal_unit=W
  C heatsink diode : fl_lib/Thermal/Thermal Elements/Thermal Mass  mass_type=foundation.enum.constant_variable.constant  mass=mass_heatsink_m kg  sp_heat=specific_heat_m J/(K*kg)  mass_min=1e-6 kg  num_ports=foundation.enum.numPorts2.one  m_specify=off  m_priority=High  m=1 kg  m_nominal_specify=off  m_nominal_value=1  m_nominal_unit=kg  T_specify=on  T_priority=High  T=Tambient_m degC  T_nominal_specify=off  T_nominal_value=1  T_nominal_unit=K  Q_specify=off  Q_priority=High  Q=0 W  Q_nominal_specify=off  Q_nominal_value=1  Q_nominal_unit=W
  Rth HA diode : fl_lib/Thermal/Thermal Elements/Thermal Resistance  resistance=rth_diode_HA_m K/W  T_specify=off  T_priority=High  T=0 deltadegC  T_nominal_specify=off  T_nominal_value=1  T_nominal_unit=K  Q_specify=off  Q_priority=None  Q=0 W  Q_nominal_specify=off  Q_nominal_value=1  Q_nominal_unit=W
  Tambient diode : fl_lib/Thermal/Thermal Sources/Temperature Source  temperature=Tambient_m degC
  dT JH diode : fl_lib/Thermal/Thermal Sensors/Temperature Sensor  temperature_measure=foundation.enum.MeasurementReference.difference
  dT HA diode : fl_lib/Thermal/Thermal Sensors/Temperature Sensor  temperature_measure=foundation.enum.MeasurementReference.difference
  dT_JH_d_K : nesl_utility/PS-Simulink Converter  PhysicalDomain=network_engine_domain  SubClassName=ps_output  LeftPortType=input  RightPortType=output  PseudoPeriodic=off  Frequencies=[]  VectorFormat=1-D array  Unit=K  AffineConversion=off
  dT_HA_d_K : nesl_utility/PS-Simulink Converter  PhysicalDomain=network_engine_domain  SubClassName=ps_output  LeftPortType=input  RightPortType=output  PseudoPeriodic=off  Frequencies=[]  VectorFormat=1-D array  Unit=K  AffineConversion=off
  i_t : Outport
  v : Outport  Port=2
  p_t : Outport  Port=3
  dT_JH_t : Outport  Port=4
  dT_HA_t : Outport  Port=5
  i_d : Outport  Port=6
  p_d : Outport  Port=7
  dT_JH_d : Outport  Port=8
  dT_HA_d : Outport  Port=9
  wires:
  i_t_A/1 -> i_t/1
  v_V/1 -> v/1
  p_t_W/1 -> p_t/1
  dT_JH_t_K/1 -> dT_JH_t/1
  dT_HA_t_K/1 -> dT_HA_t/1
  i_d_A/1 -> i_d/1
  p_d_W/1 -> p_d/1
  dT_JH_d_K/1 -> dT_JH_d/1
  dT_HA_d_K/1 -> dT_HA_d/1
  g/1 -> gate/1
  connections:
  Rth JH transistor/RConn1 -- C heatsink transistor/LConn1 -- Rth HA transistor/LConn1 -- dT JH transistor/RConn1 -- dT HA transistor/LConn1
  Rth HA transistor/RConn1 -- Tambient transistor/LConn1 -- dT HA transistor/RConn1
  dT JH transistor/RConn2 -- dT_JH_t_K/LConn1
  dT HA transistor/RConn2 -- dT_HA_t_K/LConn1
  Rth JH diode/RConn1 -- C heatsink diode/LConn1 -- Rth HA diode/LConn1 -- dT JH diode/RConn1 -- dT HA diode/LConn1
  Rth HA diode/RConn1 -- Tambient diode/LConn1 -- dT HA diode/RConn1
  dT JH diode/RConn2 -- dT_JH_d_K/LConn1
  dT HA diode/RConn2 -- dT_HA_d_K/LConn1
  gate/RConn1 -- mos_simple_2th/LConn3
  D/RConn1 -- mos_simple_2th/LConn1 -- RC snubber/LConn1 -- v_sensor/LConn1
  mos_simple_2th/RConn1 -- S/RConn1 -- RC snubber/RConn1 -- v_sensor/RConn2
  v_sensor/RConn1 -- v_V/LConn1
  mos_simple_2th/RConn3 -- p_t_W/LConn1
  mos_simple_2th/RConn4 -- p_d_W/LConn1
  mos_simple_2th/RConn5 -- i_t_A/LConn1
  mos_simple_2th/RConn6 -- i_d_A/LConn1
  mos_simple_2th/LConn2 -- Cj transistor/LConn1 -- Rth JH transistor/LConn1 -- dT JH transistor/LConn1
  mos_simple_2th/RConn2 -- Cj diode/LConn1 -- Rth JH diode/LConn1 -- dT JH diode/LConn1

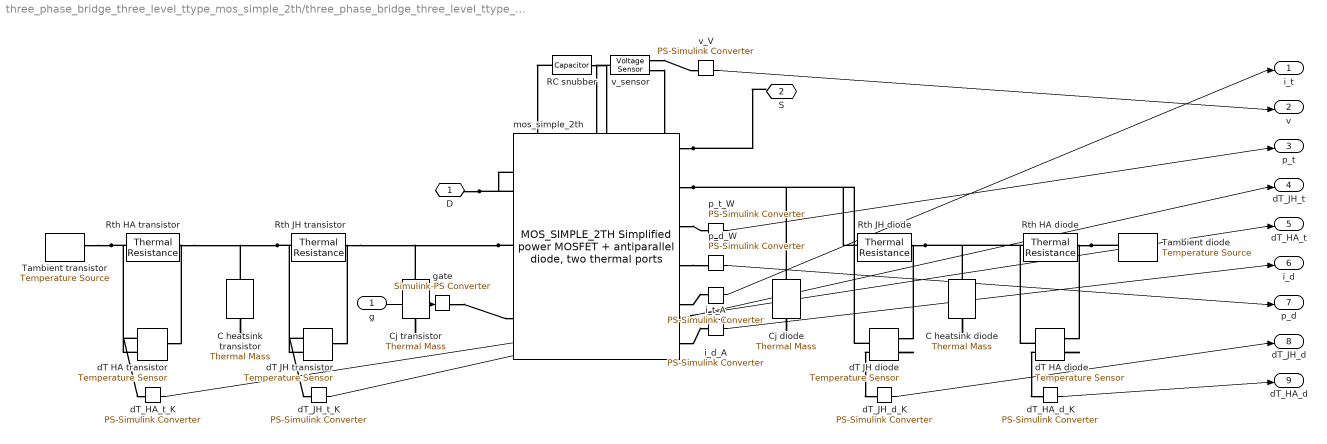
== system three_phase_bridge_three_level_ttype_mos_simple_2th/three_phase_bridge_three_level_ttype_mos_simple_2th/Q7 ==
  g : Inport
  gate : nesl_utility/Simulink-PS Converter  PhysicalDomain=network_engine_domain  SubClassName=ps_input  LeftPortType=input  RightPortType=output  PseudoPeriodic=off  Frequencies=[]  NoiseDistribution=none  NoiseParameters=[]  Unit=1  AffineConversion=off  FilteringAndDerivatives=provide  SimscapeFilterOrder=1  InputFilterTimeConstant=0.001  UdotUserProvided=0
  mos_simple_2th : mos_simple_2th_lib/MOS_SIMPLE_2TH Simplified power MOSFET + antiparallel diode, two thermal ports  Rds_on=rds_on_m mOhm  alpha_R=alpha_R_m 1/K  Tj_ref=Tj_ref_m degC  Roff=Roff_m Ohm  Vf=v_gamma_m V  Rd=rd_on_m mOhm  two_die=two_die_m  G_th=G_th_m  Eon_ref=Eon_m mJ  Eoff_ref=Eoff_m mJ  Err_ref=Err_m mJ  Iref=Ic_ref_m A  Vref=Vdc_ref_m V  ki=ki_m  kv=kv_m  Vth_off=Vth_off_m V  Vth_on=Vth_on_m V  V_sm=V_sm_m V  tau_s=time_constant_edge_m us  tau_v=tau_v_m us  tau_p=time_constant_ploss_m us  i_eps=i_eps_m A  v_eps=1e-3 V  v_specify=off  v_priority=None  v=0 V  v_nominal_specify=off  v_nominal_value=1  v_nominal_unit=V  i_specify=off  i_priority=None  i=0 A  i_nominal_specify=off  i_nominal_value=1  i_nominal_unit=A  ich_specify=off  ich_priority=None  ich=0 A  ich_nominal_specify=off  ich_nominal_value=1  ich_nominal_unit=A  ichp_specify=off  ichp_priority=None  ichp=0 A  ichp_nominal_specify=off  ichp_nominal_value=1  ichp_nominal_unit=A  idio_specify=off  idio_priority=None  idio=0 A  idio_nominal_specify=off  idio_nominal_value=1  idio_nominal_unit=A  vfd_specify=off  vfd_priority=None  vfd=0 V  vfd_nominal_specify=off  vfd_nominal_value=1  vfd_nominal_unit=V  ith_specify=off  ith_priority=None  ith=0 A  ith_nominal_specify=off  ith_nominal_value=1  ith_nominal_unit=A  idh_specify=off  idh_priority=None  idh=0 A  idh_nominal_specify=off  idh_nominal_value=1  idh_nominal_unit=A  vbl_specify=off  vbl_priority=None  vbl=600 V  vbl_nominal_specify=off  vbl_nominal_value=1  vbl_nominal_unit=V  hb_specify=off  hb_priority=None  hb=0  hb_nominal_specify=off  hb_nominal_value=1  hb_nominal_unit=1  Gch_specify=off  Gch_priority=None  Gch=0 S  Gch_nominal_specify=off  Gch_nominal_value=1  Gch_nominal_unit=S  gl_specify=off  gl_priority=None  gl=0  gl_nominal_specify=off  gl_nominal_value=1  gl_nominal_unit=1  Rds_specify=off  Rds_priority=None  Rds=1e-3 Ohm  Rds_nominal_specify=off  Rds_nominal_value=1  Rds_nominal_unit=Ohm  xr_specify=off  xr_priority=None  xr=1  xr_nominal_specify=off  xr_nominal_value=1  xr_nominal_unit=1  Eot_specify=off  Eot_priority=None  Eot=0 J  Eot_nominal_specify=off  Eot_nominal_value=1  Eot_nominal_unit=J  Eod_specify=off  Eod_priority=None  Eod=0 J  Eod_nominal_specify=off  Eod_nominal_value=1  Eod_nominal_unit=J  Pswt_specify=off  Pswt_priority=None  Pswt=0 W  Pswt_nominal_specify=off  Pswt_nominal_value=1  Pswt_nominal_unit=W  Pswd_specify=off  Pswd_priority=None  Pswd=0 W  Pswd_nominal_specify=off  Pswd_nominal_value=1  Pswd_nominal_unit=W  Pct_specify=off  Pct_priority=None  Pct=0 W  Pct_nominal_specify=off  Pct_nominal_value=1  Pct_nominal_unit=W  Pcd_specify=off  Pcd_priority=None  Pcd=0 W  Pcd_nominal_specify=off  Pcd_nominal_value=1  Pcd_nominal_unit=W  Qt_specify=off  Qt_priority=None  Qt=0 W  Qt_nominal_specify=off  Qt_nominal_value=1  Qt_nominal_unit=W  Qd_specify=off  Qd_priority=None  Qd=0 W  Qd_nominal_specify=off  Qd_nominal_value=1  Qd_nominal_unit=W  Eqt_specify=off  Eqt_priority=None  Eqt=0 J  Eqd_specify=off  Eqd_priority=None  Eqd=0 J
  D : PMIOPort  Side=Left
  S : PMIOPort  Port=2  Side=Right
  RC snubber : fl_lib/Electrical/Electrical Elements/Capacitor  c=Csnubber_m F  r=Rsnubber_m Ohm  g=0 1/Ohm  i_specify=off  i_priority=None  i=0 A  i_nominal_specify=off  i_nominal_value=1  i_nominal_unit=A  v_specify=off  v_priority=None  v=0 V  v_nominal_specify=off  v_nominal_value=1  v_nominal_unit=V  vc_specify=off  vc_priority=High  vc=0 V  vc_nominal_specify=off  vc_nominal_value=1  vc_nominal_unit=V
  v_sensor : fl_lib/Electrical/Electrical Sensors/Voltage Sensor
  v_V : nesl_utility/PS-Simulink Converter  PhysicalDomain=network_engine_domain  SubClassName=ps_output  LeftPortType=input  RightPortType=output  PseudoPeriodic=off  Frequencies=[]  VectorFormat=1-D array  Unit=V  AffineConversion=off
  p_t_W : nesl_utility/PS-Simulink Converter  PhysicalDomain=network_engine_domain  SubClassName=ps_output  LeftPortType=input  RightPortType=output  PseudoPeriodic=off  Frequencies=[]  VectorFormat=1-D array  Unit=W  AffineConversion=off
  p_d_W : nesl_utility/PS-Simulink Converter  PhysicalDomain=network_engine_domain  SubClassName=ps_output  LeftPortType=input  RightPortType=output  PseudoPeriodic=off  Frequencies=[]  VectorFormat=1-D array  Unit=W  AffineConversion=off
  i_t_A : nesl_utility/PS-Simulink Converter  PhysicalDomain=network_engine_domain  SubClassName=ps_output  LeftPortType=input  RightPortType=output  PseudoPeriodic=off  Frequencies=[]  VectorFormat=1-D array  Unit=A  AffineConversion=off
  i_d_A : nesl_utility/PS-Simulink Converter  PhysicalDomain=network_engine_domain  SubClassName=ps_output  LeftPortType=input  RightPortType=output  PseudoPeriodic=off  Frequencies=[]  VectorFormat=1-D array  Unit=A  AffineConversion=off
  Cj transistor : fl_lib/Thermal/Thermal Elements/Thermal Mass  mass_type=foundation.enum.constant_variable.constant  mass=JunctionTermalMass_m/specific_heat_m kg  sp_heat=specific_heat_m J/(K*kg)  mass_min=1e-6 kg  num_ports=foundation.enum.numPorts2.one  m_specify=off  m_priority=High  m=1 kg  m_nominal_specify=off  m_nominal_value=1  m_nominal_unit=kg  T_specify=on  T_priority=High  T=Tambient_m degC  T_nominal_specify=off  T_nominal_value=1  T_nominal_unit=K  Q_specify=off  Q_priority=High  Q=0 W  Q_nominal_specify=off  Q_nominal_value=1  Q_nominal_unit=W
  Rth JH transistor : fl_lib/Thermal/Thermal Elements/Thermal Resistance  resistance=rth_switch_JH_m K/W  T_specify=off  T_priority=High  T=0 deltadegC  T_nominal_specify=off  T_nominal_value=1  T_nominal_unit=K  Q_specify=off  Q_priority=None  Q=0 W  Q_nominal_specify=off  Q_nominal_value=1  Q_nominal_unit=W
  C heatsink transistor : fl_lib/Thermal/Thermal Elements/Thermal Mass  mass_type=foundation.enum.constant_variable.constant  mass=mass_heatsink_m kg  sp_heat=specific_heat_m J/(K*kg)  mass_min=1e-6 kg  num_ports=foundation.enum.numPorts2.one  m_specify=off  m_priority=High  m=1 kg  m_nominal_specify=off  m_nominal_value=1  m_nominal_unit=kg  T_specify=on  T_priority=High  T=Tambient_m degC  T_nominal_specify=off  T_nominal_value=1  T_nominal_unit=K  Q_specify=off  Q_priority=High  Q=0 W  Q_nominal_specify=off  Q_nominal_value=1  Q_nominal_unit=W
  Rth HA transistor : fl_lib/Thermal/Thermal Elements/Thermal Resistance  resistance=rth_switch_HA_m K/W  T_specify=off  T_priority=High  T=0 deltadegC  T_nominal_specify=off  T_nominal_value=1  T_nominal_unit=K  Q_specify=off  Q_priority=None  Q=0 W  Q_nominal_specify=off  Q_nominal_value=1  Q_nominal_unit=W
  Tambient transistor : fl_lib/Thermal/Thermal Sources/Temperature Source  temperature=Tambient_m degC
  dT JH transistor : fl_lib/Thermal/Thermal Sensors/Temperature Sensor  temperature_measure=foundation.enum.MeasurementReference.difference
  dT HA transistor : fl_lib/Thermal/Thermal Sensors/Temperature Sensor  temperature_measure=foundation.enum.MeasurementReference.difference
  dT_JH_t_K : nesl_utility/PS-Simulink Converter  PhysicalDomain=network_engine_domain  SubClassName=ps_output  LeftPortType=input  RightPortType=output  PseudoPeriodic=off  Frequencies=[]  VectorFormat=1-D array  Unit=K  AffineConversion=off
  dT_HA_t_K : nesl_utility/PS-Simulink Converter  PhysicalDomain=network_engine_domain  SubClassName=ps_output  LeftPortType=input  RightPortType=output  PseudoPeriodic=off  Frequencies=[]  VectorFormat=1-D array  Unit=K  AffineConversion=off
  Cj diode : fl_lib/Thermal/Thermal Elements/Thermal Mass  mass_type=foundation.enum.constant_variable.constant  mass=JunctionTermalMass_m/specific_heat_m kg  sp_heat=specific_heat_m J/(K*kg)  mass_min=1e-6 kg  num_ports=foundation.enum.numPorts2.one  m_specify=off  m_priority=High  m=1 kg  m_nominal_specify=off  m_nominal_value=1  m_nominal_unit=kg  T_specify=on  T_priority=High  T=Tambient_m degC  T_nominal_specify=off  T_nominal_value=1  T_nominal_unit=K  Q_specify=off  Q_priority=High  Q=0 W  Q_nominal_specify=off  Q_nominal_value=1  Q_nominal_unit=W
  Rth JH diode : fl_lib/Thermal/Thermal Elements/Thermal Resistance  resistance=rth_diode_JH_m K/W  T_specify=off  T_priority=High  T=0 deltadegC  T_nominal_specify=off  T_nominal_value=1  T_nominal_unit=K  Q_specify=off  Q_priority=None  Q=0 W  Q_nominal_specify=off  Q_nominal_value=1  Q_nominal_unit=W
  C heatsink diode : fl_lib/Thermal/Thermal Elements/Thermal Mass  mass_type=foundation.enum.constant_variable.constant  mass=mass_heatsink_m kg  sp_heat=specific_heat_m J/(K*kg)  mass_min=1e-6 kg  num_ports=foundation.enum.numPorts2.one  m_specify=off  m_priority=High  m=1 kg  m_nominal_specify=off  m_nominal_value=1  m_nominal_unit=kg  T_specify=on  T_priority=High  T=Tambient_m degC  T_nominal_specify=off  T_nominal_value=1  T_nominal_unit=K  Q_specify=off  Q_priority=High  Q=0 W  Q_nominal_specify=off  Q_nominal_value=1  Q_nominal_unit=W
  Rth HA diode : fl_lib/Thermal/Thermal Elements/Thermal Resistance  resistance=rth_diode_HA_m K/W  T_specify=off  T_priority=High  T=0 deltadegC  T_nominal_specify=off  T_nominal_value=1  T_nominal_unit=K  Q_specify=off  Q_priority=None  Q=0 W  Q_nominal_specify=off  Q_nominal_value=1  Q_nominal_unit=W
  Tambient diode : fl_lib/Thermal/Thermal Sources/Temperature Source  temperature=Tambient_m degC
  dT JH diode : fl_lib/Thermal/Thermal Sensors/Temperature Sensor  temperature_measure=foundation.enum.MeasurementReference.difference
  dT HA diode : fl_lib/Thermal/Thermal Sensors/Temperature Sensor  temperature_measure=foundation.enum.MeasurementReference.difference
  dT_JH_d_K : nesl_utility/PS-Simulink Converter  PhysicalDomain=network_engine_domain  SubClassName=ps_output  LeftPortType=input  RightPortType=output  PseudoPeriodic=off  Frequencies=[]  VectorFormat=1-D array  Unit=K  AffineConversion=off
  dT_HA_d_K : nesl_utility/PS-Simulink Converter  PhysicalDomain=network_engine_domain  SubClassName=ps_output  LeftPortType=input  RightPortType=output  PseudoPeriodic=off  Frequencies=[]  VectorFormat=1-D array  Unit=K  AffineConversion=off
  i_t : Outport
  v : Outport  Port=2
  p_t : Outport  Port=3
  dT_JH_t : Outport  Port=4
  dT_HA_t : Outport  Port=5
  i_d : Outport  Port=6
  p_d : Outport  Port=7
  dT_JH_d : Outport  Port=8
  dT_HA_d : Outport  Port=9
  wires:
  i_t_A/1 -> i_t/1
  v_V/1 -> v/1
  p_t_W/1 -> p_t/1
  dT_JH_t_K/1 -> dT_JH_t/1
  dT_HA_t_K/1 -> dT_HA_t/1
  i_d_A/1 -> i_d/1
  p_d_W/1 -> p_d/1
  dT_JH_d_K/1 -> dT_JH_d/1
  dT_HA_d_K/1 -> dT_HA_d/1
  g/1 -> gate/1
  connections:
  Rth JH transistor/RConn1 -- C heatsink transistor/LConn1 -- Rth HA transistor/LConn1 -- dT JH transistor/RConn1 -- dT HA transistor/LConn1
  Rth HA transistor/RConn1 -- Tambient transistor/LConn1 -- dT HA transistor/RConn1
  dT JH transistor/RConn2 -- dT_JH_t_K/LConn1
  dT HA transistor/RConn2 -- dT_HA_t_K/LConn1
  Rth JH diode/RConn1 -- C heatsink diode/LConn1 -- Rth HA diode/LConn1 -- dT JH diode/RConn1 -- dT HA diode/LConn1
  Rth HA diode/RConn1 -- Tambient diode/LConn1 -- dT HA diode/RConn1
  dT JH diode/RConn2 -- dT_JH_d_K/LConn1
  dT HA diode/RConn2 -- dT_HA_d_K/LConn1
  gate/RConn1 -- mos_simple_2th/LConn3
  D/RConn1 -- mos_simple_2th/LConn1 -- RC snubber/LConn1 -- v_sensor/LConn1
  mos_simple_2th/RConn1 -- S/RConn1 -- RC snubber/RConn1 -- v_sensor/RConn2
  v_sensor/RConn1 -- v_V/LConn1
  mos_simple_2th/RConn3 -- p_t_W/LConn1
  mos_simple_2th/RConn4 -- p_d_W/LConn1
  mos_simple_2th/RConn5 -- i_t_A/LConn1
  mos_simple_2th/RConn6 -- i_d_A/LConn1
  mos_simple_2th/LConn2 -- Cj transistor/LConn1 -- Rth JH transistor/LConn1 -- dT JH transistor/LConn1
  mos_simple_2th/RConn2 -- Cj diode/LConn1 -- Rth JH diode/LConn1 -- dT JH diode/LConn1
